simulink model "coffee_machine_interactive"  (R2025b)
settings: Solver=FixedStepDiscrete  StartTime=0.0  StopTime=inf  FixedStep=0.01  RelTol=1e-3
settings Model: Creator=HP  LastModifiedBy=HP

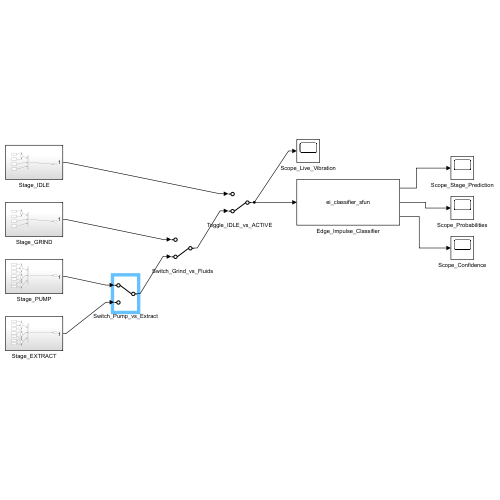
[thumbnail: Simulink's stored preview of the top-level diagram]
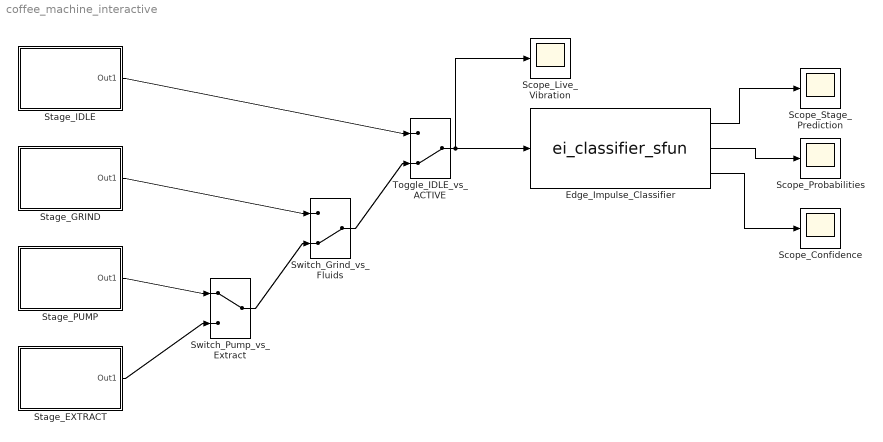
== system coffee_machine_interactive ==
  Edge_Impulse_Classifier : S-Function  FunctionName=ei_classifier_sfun  Parameters=0.01, 10  SFunctionDeploymentMode=off  EnableBusSupport=off
  Scope_Confidence : Scope
  Scope_Live_Vibration : Scope
      settings: ActiveDisplayYMinimum=-1.4108202107410153  ActiveDisplayYMaximum=11.177087801615423
  Scope_Probabilities : Scope
  Scope_Stage_Prediction : Scope
  Stage_EXTRACT : Subsystem
  Stage_GRIND : Subsystem
  Stage_IDLE : Subsystem
  Stage_PUMP : Subsystem
  Switch_Grind_vs_Fluids : ManualSwitch  CurrentSetting=0
  Switch_Pump_vs_Extract : ManualSwitch
  Toggle_IDLE_vs_ACTIVE : ManualSwitch  CurrentSetting=0
  wires:
  Stage_PUMP/1(Out1) -> Switch_Pump_vs_Extract/1
  Stage_EXTRACT/1(Out1) -> Switch_Pump_vs_Extract/2
  Stage_GRIND/1(Out1) -> Switch_Grind_vs_Fluids/1
  Switch_Pump_vs_Extract/1 -> Switch_Grind_vs_Fluids/2
  Stage_IDLE/1(Out1) -> Toggle_IDLE_vs_ACTIVE/1
  Switch_Grind_vs_Fluids/1 -> Toggle_IDLE_vs_ACTIVE/2
  Toggle_IDLE_vs_ACTIVE/1 -> Edge_Impulse_Classifier/1, Scope_Live_Vibration/1
  Edge_Impulse_Classifier/1 -> Scope_Stage_Prediction/1
  Edge_Impulse_Classifier/2 -> Scope_Probabilities/1
  Edge_Impulse_Classifier/3 -> Scope_Confidence/1

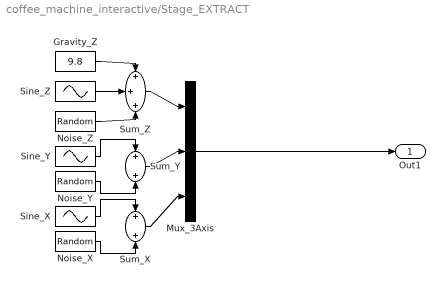
== system coffee_machine_interactive/Stage_EXTRACT ==
  Gravity_Z : Constant  Value=9.8  SampleTime=0.01
  Mux_3Axis : Mux  Inputs=3
  Noise_X : RandomNumber  Variance=0.09  SampleTime=0.01
  Noise_Y : RandomNumber  Variance=0.09  SampleTime=0.01
  Noise_Z : RandomNumber  Variance=0.16  SampleTime=0.01
  Sine_X : Sin  Amplitude=0.6  Frequency=2*pi*25  SampleTime=0.01
  Sine_Y : Sin  Amplitude=0.8  Frequency=2*pi*50  Phase=pi/2  SampleTime=0.01
  Sine_Z : Sin  Amplitude=1.2  Frequency=2*pi*50  SampleTime=0.01
  Sum_X : Sum
  Sum_Y : Sum
  Sum_Z : Sum  Inputs=+++
  Out1 : Outport
  wires:
  Gravity_Z/1 -> Sum_Z/1
  Sine_Z/1 -> Sum_Z/2
  Noise_Z/1 -> Sum_Z/3
  Sine_Y/1 -> Sum_Y/1
  Noise_Y/1 -> Sum_Y/2
  Sine_X/1 -> Sum_X/1
  Noise_X/1 -> Sum_X/2
  Sum_Z/1 -> Mux_3Axis/1
  Sum_Y/1 -> Mux_3Axis/2
  Sum_X/1 -> Mux_3Axis/3
  Mux_3Axis/1 -> Out1/1

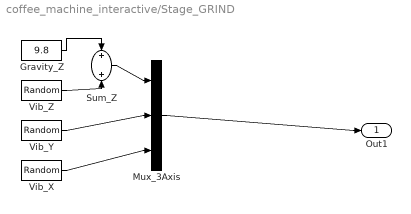
== system coffee_machine_interactive/Stage_GRIND ==
  Gravity_Z : Constant  Value=9.8  SampleTime=0.01
  Mux_3Axis : Mux  Inputs=3
  Sum_Z : Sum
  Vib_X : RandomNumber  Variance=25.0  SampleTime=0.01
  Vib_Y : RandomNumber  Variance=36.0  SampleTime=0.01
  Vib_Z : RandomNumber  Variance=64.0  SampleTime=0.01
  Out1 : Outport
  wires:
  Gravity_Z/1 -> Sum_Z/1
  Vib_Z/1 -> Sum_Z/2
  Sum_Z/1 -> Mux_3Axis/1
  Vib_Y/1 -> Mux_3Axis/2
  Vib_X/1 -> Mux_3Axis/3
  Mux_3Axis/1 -> Out1/1

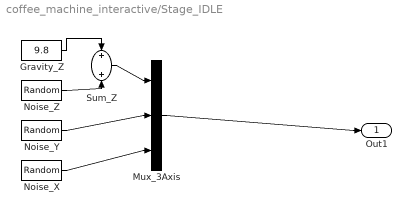
== system coffee_machine_interactive/Stage_IDLE ==
  Gravity_Z : Constant  Value=9.8  SampleTime=0.01
  Mux_3Axis : Mux  Inputs=3
  Noise_X : RandomNumber  Variance=0.0025  SampleTime=0.01
  Noise_Y : RandomNumber  Variance=0.0025  SampleTime=0.01
  Noise_Z : RandomNumber  Variance=0.0025  SampleTime=0.01
  Sum_Z : Sum
  Out1 : Outport
  wires:
  Gravity_Z/1 -> Sum_Z/1
  Noise_Z/1 -> Sum_Z/2
  Sum_Z/1 -> Mux_3Axis/1
  Noise_Y/1 -> Mux_3Axis/2
  Noise_X/1 -> Mux_3Axis/3
  Mux_3Axis/1 -> Out1/1

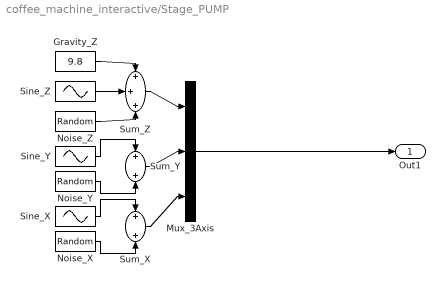
== system coffee_machine_interactive/Stage_PUMP ==
  Gravity_Z : Constant  Value=9.8  SampleTime=0.01
  Mux_3Axis : Mux  Inputs=3
  Noise_X : RandomNumber  Variance=0.04  SampleTime=0.01
  Noise_Y : RandomNumber  Variance=0.04  SampleTime=0.01
  Noise_Z : RandomNumber  Variance=0.09  SampleTime=0.01
  Sine_X : Sin  Amplitude=1.2  Frequency=2*pi*25  SampleTime=0.01
  Sine_Y : Sin  Amplitude=1.8  Frequency=2*pi*50  Phase=pi/2  SampleTime=0.01
  Sine_Z : Sin  Amplitude=2.5  Frequency=2*pi*50  SampleTime=0.01
  Sum_X : Sum
  Sum_Y : Sum
  Sum_Z : Sum  Inputs=+++
  Out1 : Outport
  wires:
  Gravity_Z/1 -> Sum_Z/1
  Sine_Z/1 -> Sum_Z/2
  Noise_Z/1 -> Sum_Z/3
  Sine_Y/1 -> Sum_Y/1
  Noise_Y/1 -> Sum_Y/2
  Sine_X/1 -> Sum_X/1
  Noise_X/1 -> Sum_X/2
  Sum_Z/1 -> Mux_3Axis/1
  Sum_Y/1 -> Mux_3Axis/2
  Sum_X/1 -> Mux_3Axis/3
  Mux_3Axis/1 -> Out1/1
